simulink library "sm_wheel_loader_lib"  (R2025a)
settings: Solver=VariableStepAuto  StartTime=0.0  StopTime=10.0  RelTol=1e-3
undefined symbols (not defined in the file): AToTOrificeVector, BiPOrificeVector, boomHEArea, boomREArea, BToTOrificeVector, fluids, GRake, GToothL, GToothR, HMPST, HydFcnParams, logLoad, Position, PToAOrificeVector, PToBOrificeVector, RakeL, RakeR, testInput, Wheel_Loader, X, Y, Z
libraries: sm_lib x694, fl_lib x183, nesl_utility x74, SimscapeFluids_lib x62, sdl_lib x25, cvt_components_lib x25, simulink_extras x5, $bdroot x4, wheel_loader_contact_lib x4, ee_lib x2, SignalEditorBlockLib x1, batteryecm_lib x1
(part 2 of 26)

== system sm_wheel_loader_lib/Engine Generic ==
  EngCtrl : Inport
  Acc to I Gain : Lookup_n-D  NumberOfTableDimensions=1  BreakpointsForDimension1=[-2 -1 0 1 2]  Table=[25 25 15 15 15]  InternalRulePriority=Speed  RndMeth=Simplest
  Acc to P Gain : Lookup_n-D  NumberOfTableDimensions=1  BreakpointsForDimension1=[-2 -1 0 1 2]  Table=[50 50 15 15 15]  InternalRulePriority=Speed  RndMeth=Simplest
  Add : Sum  Inputs=+-
  Bus Creator : BusCreator  Inputs=2
  Bus Selector : BusSelector  OutputSignals=CmdEngSpd(RPM),CmdSpdRate
  Generic Engine : sdl_lib/Engines & Motors/Generic Engine  input_type=sdl.enum.GenericEngineInputType.TorqueCommand  model_parameterization=sdl.enum.engineParameterization.torque  engine_type=sdl.enum.engineType.SI  Trq_max=380 N*m  w_Trq_max=4300 rpm  P_max=230 kW  w_P_max=6858 rpm  w_max=7000 rpm  w_min=500 rpm  w_tab=[HMPST.Eng.MaxTorq.SpdVec(2:end) 3000] rpm  trq_tab=[HMPST.Eng.MaxTorq.TrqVec(2:end-2) 10 10 10] N*m  pwr_tab=[10, 30, 70, 110, 165, 190, 220, 230] kW  interp_method=simscape.enum.interpolation.linear  w_thr=100 rpm  model_inertia=sdl.enum.model_inertia.on  inertia=1 kg*m^2  initial_velocity=HMPST.Eng.wTarget rpm  model_time_constant=sdl.enum.lagOffOn.off  time_constant=0.2 s  initial_normalized_throttle=0  fc_model=sdl.enum.fuel_consumption_model.FuelOff  fc_per_rev=25 mg/rev  fc_w_tab=[1000, 2000, 3000, 4000, 5000, 6000] rpm  fc_trq_tab=[0, 80, 160, 200, 240, 320, 360, 400] N*m  fc_tab=[.5, .9, 1.4, 1.6, 1.9, 2.7, 3.4, 4.4; 1, 1.7, 2.7, 3.1, 3.6, 5, 6, 7.4; 1.4, 2.7, 4, 4.8, 5.6, 7.5, 8.5, 10.5; 2, 3.6, 5.8, 6.7, 8, 10.4, 11.7, 13.3; 2.5, 4.8, 7.9, 9.4, 10.8, 14, 16.2, 18.6; 3.1, 6, 10.3, 11.9, 13.8, 18.4, 22, 26.5] g/s  bmep_tab=[0, 250, 500, 625, 750, 1000, 1150, 1250] kPa  bsfc_tab=[410, 380, 300, 280, 270, 290, 320, 380; 410, 370, 290, 270, 260, 270, 285, 320; 415, 380, 290, 275, 265, 270, 270, 300; 420, 390, 310, 290, 285, 280, 280, 285; 430, 410, 340, 320, 310, 300, 310, 320; 450, 430, 370, 340, 330, 330, 350, 380] g/(hr*kW)  fc_interp_method=simscape.enum.interpolation.linear  displaced_volume=400 cm^3  rev_per_cycle=2  idle_speed=false  idle_speed_reference=1000 rpm  tau_controller=1 s  idle_w_thr=1 rpm  redline=false  redline_speed=5000 rpm  tau_redline=1 s  redline_w_thr=1 rpm
      settings: InternalSimscapePortConfiguration="{\"Bottom\":[],\"Left\":[{\"id\":\"TrqCmd\",\"label\":\"Trq\",\"type\":\"input\"},{\"id\":\"B\",\"label\":\"B\",\"type\":\"foundation.mechanical.rotational.rotational\"}],\"Right\":[{\"id\":\"P\",\"label\":\"P\",\"type\":\"output\"},{\"id\":\"FC\",\"label\":\"FC\",\"type\":\"output\"},{\"id\":\"F\",\"label\":\"F\",\"type\":\"foundation.mechanical.rotational.rotational\"}],\"Top\":[]}"
  Mechanical Rotational Reference : fl_lib/Mechanical/Rotational Elements/Mechanical Rotational Reference
  PID Controller : slpidlib/PID Controller  Controller=PI  Form=Parallel  TimeDomain=Continuous-time  UseExternalTs=off  SampleTime=-1  IntegratorMethod=Forward Euler  FilterMethod=Forward Euler  ControllerParametersSource=external  P=15  I=10  UseKiTs=off  D=0  UseExternalDerivativeSource=off  N=100  UseFilter=on  TunerSelectOption=Transfer Function Based (PID Tuner App)  InitialConditionSource=internal  InitialConditionForIntegrator=0  InitialConditionForFilter=0  DifferentiatorICPrevScaledInput=0  ExternalReset=none  TrackingMode=on  Kt=100  LimitOutput=off  SatLimitsSource=internal  UpperSaturationLimit=inf  LowerSaturationLimit=-inf  LinearizeAsGain=on  AntiWindupMode=none  Kb=1  LimitIntegrator=off  UpperIntegratorSaturationLimit=inf  LowerIntegratorSaturationLimit=-inf  POutMin=[]  POutMax=[]  IOutMin=[]  IOutMax=[]  DOutMin=[]  DOutMax=[]  NOutMin=[]  NOutMax=[]  SumOutMin=[]  SumOutMax=[]  SaturationOutMin=[]  SaturationOutMax=[]  PParamMin=[]  PParamMax=[]  IParamMin=[]  IParamMax=[]  DParamMin=[]  DParamMax=[]  NParamMin=[]  NParamMax=[]  KbParamMin=[]  KbParamMax=[]  KtParamMin=[]  KtParamMax=[]  KbOutMin=[]  KbOutMax=[]  KtOutMin=[]  KtOutMax=[]  IntegratorOutMin=[]  IntegratorOutMax=[]  FilterOutMin=[]  FilterOutMax=[]  SumI1OutMin=[]  SumI1OutMax=[]  SumI2OutMin=[]  SumI2OutMax=[]  SumI3OutMin=[]  SumI3OutMax=[]  SumI4OutMin=[]  SumI4OutMax=[]  SumDOutMin=[]  SumDOutMax=[]  DifferentiatorOutMin=[]  DifferentiatorOutMax=[]  FilterDiffOutCoefMin=[]  FilterDiffOutCoefMax=[]  ReciprocalOutMin=[]  ReciprocalOutMax=[]  SumDenOutMin=[]  SumDenOutMax=[]  SumNumOutMin=[]  SumNumOutMax=[]  DivideOutMin=[]  DivideOutMax=[]  UdiffTsProdOutMin=[]  UdiffTsProdOutMax=[]  NTsProdOutMin=[]  NTsProdOutMax=[]  UintegralTsProdOutMin=[]  UintegralTsProdOutMax=[]  UngainTsProdOutMin=[]  UngainTsProdOutMax=[]  ClampingZeroOutDataTypeStr=Inherit: Inherit via back propagation  ClampingZeroOutMin=[]  ClampingZeroOutMax=[]  FilterDenConstantOutDataTypeStr=Inherit: Inherit via back propagation  FilterDenConstantOutMin=[]  FilterDenConstantOutMax=[]  PCopyOutDataTypeStr=Inherit: Inherit via back propagation  PCopyOutMin=[]  PCopyOutMax=[]  NCopyOutDataTypeStr=Inherit: Inherit via back propagation  NCopyOutMin=[]  NCopyOutMax=[]  IntegratorContinuousStateAttributes=''  IntegratorStateMustResolveToSignalObject=off  IntegratorRTWStateStorageClass=Auto  FilterContinuousStateAttributes=''  FilterStateMustResolveToSignalObject=off  FilterRTWStateStorageClass=Auto  ParallelPVariant=ExternalParameters  IdealPVariant=Disabled  IVariant=ExternalParameters  DVariant=Disabled  IntegratorVariant=Continuous  SatVariant=Disabled  AWVariant=Passthrough  PCopyVariant=Disabled  TRVariant=Enabled  FdbkBlocksVariant=Forward  IdealPFdbkVariant=Disabled  SatFdbkVariant=Disabled  DerivativeFilterVariant=Disabled  NVariant=Disabled  NCopyVariant=Disabled_SignalSpec  FilterICVariant=Disabled  IntegratorICVariant=InternalICs  ExternalResetVariant=Disabled  TRSumVariant=TrackingMode  SumFdbkVariant=Disabled  SumVariant=Sum_PI  TsampFilterVariant=InternalTs  TsampNgainVariant=Passthrough  TsampIntegralVariant=Disabled_SignalSpec  ExternalSaturationOutDataTypeStr=Inherit: Same as second input  DerivativeSourceVariant=Disabled  PreIntVariant=InternalPreInt
  Simulink-PS Converter : nesl_utility/Simulink-PS Converter  PhysicalDomain=network_engine_domain  SubClassName=ps_input  LeftPortType=input  RightPortType=output  PseudoPeriodic=off  Frequencies=[]  NoiseDistribution=none  NoiseParameters=[]  Unit=1  AffineConversion=off  FilteringAndDerivatives=provide  SimscapeFilterOrder=1  InputFilterTimeConstant=0.001  UdotUserProvided=0
  Speed Sensor : Subsystem
  Subsystem : Subsystem
      settings: PortSchema="{\"entries\":[{\"content\":{\"sides\":[{\"content\":{\"connectorIds\":[\"LConn1\"]},\"type\":\"ConnectorPlacement.EquallySpacedRectSide\",\"uuid\":\"5a764f16-cafe-4867-b916-6b4e7e02daa5\"},{\"content\":{\"connectorIds\":[\"RConn1\"],\"side\":\"RIGHT\"},\"type\":\"ConnectorPlacement.EquallySpacedRectSide\",\"uuid\":\"8ceee8ac-f09f-4a1d-836f-79964ce3b2d4\"},{\"content\":{\"connectorIds\":[\"Out1\"],\"side\":\"TOP\"},\"type\":\"ConnectorPlacement.EquallySpacedRectSide\",\"uuid\":\"effcec0c-0a3a-409b-822c-5f5bf6cd9579\"}]},\"type\":\"ConnectorPlacement.EquallySpacedConnector\",\"uuid\":\"cbc631ce-3260-4296-836f-4219c3ba8d3a\"}],\"packageUris\":[\"http://schema.mathworks.com/mf0/Connector/R2020b\"],\"version\":\"1.0\"}"
  Transfer Fcn (with initial outputs) : simulink_extras/Additional Linear/Transfer Fcn (with initial outputs)  N=[1]  D="[0.1  1]"  Y0=HMPST.Eng.wTarget  U0=0
  Trq Lim Upper : Lookup_n-D  NumberOfTableDimensions=1  BreakpointsForDimension1=HMPST.Eng.MaxTorq.SpdVec  Table=HMPST.Eng.MaxTorq.TrqVec  ExtrapMethod=Clip  InternalRulePriority=Speed  RndMeth=Simplest
  Shaft : PMIOPort  Side=Right
  EngFbk : Outport
  Out Bus Element : Outport  Port=2  PortName=m  Element=w.cmd
  Out Bus Element1 : Outport  Port=2  PortName=m  Element=w.meas
  Out Bus Element2 : Outport  Port=2  PortName=m  Element=trq.limUp
  Out Bus Element3 : Outport  Port=2  PortName=m  Element=trq.meas
  Out Bus Element4 : Outport  Port=2  PortName=m  Element=trq.Cmd
  wires:
  Bus Creator/1 -> EngFbk/1
  Bus Selector/1 -> Transfer Fcn (with initial outputs)/1  "<CmdEngSpd(RPM)>"
  EngCtrl/1 -> Bus Selector/1
  Bus Selector/2 -> Acc to P Gain/1, Acc to I Gain/1  "<CmdSpdRate>"
  Acc to P Gain/1 -> PID Controller/2
  Acc to I Gain/1 -> PID Controller/3
  Speed Sensor/1(w (rpm)) -> Add/2, Out Bus Element1/1, Trq Lim Upper/1, Bus Creator/2  "ActuEngSpd(RPM)"
  Trq Lim Upper/1 -> Out Bus Element2/1  "UL_Trq"
  PID Controller/1 -> Out Bus Element4/1, PID Controller/4, Bus Creator/1, Simulink-PS Converter/1  "ActuEngTrq(Nm)"
  Transfer Fcn (with initial outputs)/1 -> Add/1, Out Bus Element/1  "Cmd Speed (RPM)"
  Add/1 -> PID Controller/1
  Subsystem/1(m) -> Out Bus Element3/1
  connections:
  Speed Sensor/LConn1 -- Subsystem/LConn1 -- Generic Engine/RConn3
  Mechanical Rotational Reference/LConn1 -- Generic Engine/LConn2
  Simulink-PS Converter/RConn1 -- Generic Engine/LConn1
  Shaft/RConn1 -- Subsystem/RConn1

== system sm_wheel_loader_lib/Hydrostatic ==
  note: Convert transmission ratio to swash plate ratio
  BusElementIn : Inport  PortName=Ctrl  Element=MBCtrl
  BusElementIn1 : Inport  PortName=Ctrl  Element=ratio
  BusElementIn2 : Inport  PortName=Ctrl  Element=CmdVehSpdDir
  Bearing Friction : sdl_lib/Couplings & Drives/Springs & Dampers/Rotational Damper  D=HMPST.Bearing.dVisc N*m*s/rad  thermal_port=simscape.enum.thermaleffects.omit  thermal_mass=50 kJ/K  temperature_specify=off  temperature_priority=High  temperature=300 K  temperature_nominal_specify=off  temperature_nominal_value=1  temperature_nominal_unit=K
  Brake Out : cvt_components_lib/Brake  bore=HMPST.Brake.cylBore  brkwy_vel=HMPST.Brake.vBrk  mu_static=HMPST.Brake.muSta  mu_coulomb=HMPST.Brake.muKin  n_pads=HMPST.Brake.numPads  r_mean=HMPST.Brake.rPad  visc_coef=HMPST.Brake.dVisc  logic2pressure=HMPST.Brake.logic2Press  ts_filt=HMPST.Brake.tsFilt
  Constant : Constant  Value=0
  Constant1 : Constant  Value=HMPST.Eng.wTarget/HMPST.HydroUnit.Pump.SpeedLimit
  Constant2 : Constant  Value=HMPST.HydroUnit.Motor.Disp/HMPST.HydroUnit.Pump.Disp
  Gain : Gain  Gain=-1
  Gears HS In : $bdroot/CVT Power Split Hydromechanical/Gears HS In  SystemSampleTime=-1  VariantActivationTime=update diagram  EmptyChoice=off  PassThrough=off  PassThroughVariantControl=(default)  EmptyChoiceVariantControl=(default)  AllowFlexibleInterface=on  Latency=0  AutoFrameSizeCalculation=off
  Hydrostatic : $bdroot/CVT Power Split Hydromechanical/Hydrostatic  pumpNomDisp=HMPST.HydroUnit.Pump.Disp  motorNomDisp=HMPST.HydroUnit.Motor.Disp  pumpNomSpd=HMPST.HydroUnit.Pump.SpeedLimit  motorNomSpd=HMPST.HydroUnit.Motor.wNominal  pumpNomVolEff=HMPST.HydroUnit.Pump.volEffNominal  motorNomVolEff=HMPST.HydroUnit.Motor.volEffNominal  pumpNomMechEff=HMPST.HydroUnit.Pump.mechEffNominal  motorNomMechEff=HMPST.HydroUnit.Motor.mechEffNominal  pumpNomPressGain=HMPST.HydroUnit.Pump.prGainNominal  motorNomPressDrop=HMPST.HydroUnit.Motor.prDropNominal  p_crack_differential=HMPST.HydroUnit.ChkV.pDiffCrack  press_max_differential=HMPST.HydroUnit.ChkV.pDiffMax  chkv_area_max=HMPST.HydroUnit.ChkV.aMax  chkv_area_leak=HMPST.HydroUnit.ChkV.aLeak  p_set_differential=HMPST.HydroUnit.PrV.pDiffSet  p_range=HMPST.HydroUnit.PrV.pRange  prv_area_max=HMPST.HydroUnit.PrV.aMax  prv_area_leak=HMPST.HydroUnit.PrV.aLeak  pipeLen=HMPST.HydroUnit.Pipes.len  pipeAreaGeo=HMPST.HydroUnit.Pipes.aGeom  pipeAreaHydr=HMPST.HydroUnit.Pipes.aHydr  chgPumpNomDisp=HMPST.HydroUnit.ChargePump.Disp  chgPumpNomMechEff=HMPST.HydroUnit.ChargePump.mechEffNominal  chgPumpNomPressGain=HMPST.HydroUnit.ChargePump.prGainNominal  chgPumpNomSpd=HMPST.HydroUnit.ChargePump.wNominal  chgPumpNomVolEff=HMPST.HydroUnit.ChargePump.volEffNominal  chgPumpChkvAleak=HMPST.HydroUnit.ChargePumpPrV.aLeak  chgPumpChkvAmax=HMPST.HydroUnit.ChargePumpPrV.aMax  chgPumpChkvPdiff=HMPST.HydroUnit.ChargePumpPrV.pDiffSet  chgPumpChkvPrange=HMPST.HydroUnit.ChargePumpPrV.pRange
  Mechanical Rotational Reference : fl_lib/Mechanical/Rotational Elements/Mechanical Rotational Reference
  Product : Product
  Product1 : Product  Inputs=3
  Sensor wIn : $bdroot/CVT Abstract/Sensor wIn  SystemSampleTime=-1  VariantActivationTime=update diagram  EmptyChoice=off  PassThrough=off  PassThroughVariantControl=(default)  EmptyChoiceVariantControl=(default)  AllowFlexibleInterface=on  Latency=0  AutoFrameSizeCalculation=off
  Sensor wOut : $bdroot/CVT Abstract/Sensor wOut  SystemSampleTime=-1  VariantActivationTime=update diagram  EmptyChoice=off  PassThrough=off  PassThroughVariantControl=(default)  EmptyChoiceVariantControl=(default)  AllowFlexibleInterface=on  Latency=0  AutoFrameSizeCalculation=off
  E : PMIOPort  Side=Left
  D : PMIOPort  Port=2  Side=Right
  Out Bus Element : Outport  PortName=m  Element=wIn
  Out Bus Element11 : Outport  PortName=m  Element=OutputShaft
  Out Bus Element12 : Outport  PortName=m  Element=P_acc
  wires:
  BusElementIn/1 -> Brake Out/1
  BusElementIn1/1 -> Product/1
  BusElementIn2/1 -> Product/2
  Product/1 -> Gain/1
  Sensor wOut/1 -> Out Bus Element11/1
  Sensor wIn/1 -> Out Bus Element/1
  Gain/1 -> Product1/1
  Product1/1 -> Hydrostatic/1
  Constant1/1 -> Product1/2
  Constant2/1 -> Product1/3
  Constant/1 -> Out Bus Element12/1  "P_acc"
  connections:
  E/RConn1 -- Gears HS In/LConn1
  D/RConn1 -- Sensor wOut/LConn1 -- Brake Out/RConn1 -- Bearing Friction/LConn1 -- Hydrostatic/RConn1
  Hydrostatic/LConn1 -- Gears HS In/RConn3
  Sensor wIn/LConn1 -- Gears HS In/RConn1
  Bearing Friction/RConn1 -- Mechanical Rotational Reference/LConn1

== system sm_wheel_loader_lib/Tires and Body 1D ==
  PS-Simulink Converter : nesl_utility/PS-Simulink Converter  PhysicalDomain=network_engine_domain  SubClassName=ps_output  LeftPortType=input  RightPortType=output  PseudoPeriodic=off  Frequencies=[]  VectorFormat=inherit  Unit=km/hr  AffineConversion=off
  Tire FL : sdl_lib/Tires & Vehicles/Tire (Magic Formula)  parameterization=sdl.enum.magic_tire_model.peak  F_z1=HMPST.TireMF1D.FA.fZrated N  F_x1=HMPST.TireMF1D.FA.fXrated N  kappa1=HMPST.TireMF1D.FA.slipRated  B_m=10  C_m=1.9  D_m=1  E_m=0.97  fz0=4000 N  p_Cx=1.685  p_Dx=[1.21, -.037]  p_Ex=[.344, .095, -.02, 0]  p_Kx=[21.51, -.163, .245]  p_Hx=[-.002, .002]  p_Vx=[0, 0]  rolling_radius_model=sdl.enum.RollingRadiusParameterization.Constant  r_e=HMPST.Tire.Rad m  r_0=0.3 m  breff=8.39  dreff=0.26  freff=0.074  q_re0=0.99  q_v1=0.008  longvl=17 m/s  cz=5e5 N/m  model_resistance=true  resistance_model=sdl.enum.rollingResistanceParameterization.constant  coeff=HMPST.TireMF1D.FA.rollingR.coeff  p_tire=250e3 Pa  alpha=-0.003  beta=0.97  coeff_a=84e-4  coeff_b=6.2e-4 s/m  coeff_c=1.6e-4 s^2/m^2  p_tire0=240e3 Pa  fz0_resistance=4000 N  vH0=16 m/s  q_Sy=[.0082, 0, .0014, .001, 0, 0, 1.08, -.5]  v_thr=HMPST.TireMF1D.FA.rollingR.vth m/s  enable_scaling_coefficients=false  lfzO=1  lcx=1  lmux=1  lex=1  lkx=1  lhx=1  lvx=1  lmy=1  model_compliance=sdl.enum.compliance.off  stiffness=1e6 N/m  damping=1000 N*s/m  model_inertia=sdl.enum.model_inertia.off  inertia=1 kg*m^2  initial_velocity=0 rad/s  vxlow=1 m/s  v_tr_thr=0.1 m/s  kpumin=-1.5  kpumax=1.5
  Tire FR : sdl_lib/Tires & Vehicles/Tire (Magic Formula)  parameterization=sdl.enum.magic_tire_model.peak  F_z1=HMPST.TireMF1D.FA.fZrated N  F_x1=HMPST.TireMF1D.FA.fXrated N  kappa1=HMPST.TireMF1D.FA.slipRated  B_m=10  C_m=1.9  D_m=1  E_m=0.97  fz0=4000 N  p_Cx=1.685  p_Dx=[1.21, -.037]  p_Ex=[.344, .095, -.02, 0]  p_Kx=[21.51, -.163, .245]  p_Hx=[-.002, .002]  p_Vx=[0, 0]  rolling_radius_model=sdl.enum.RollingRadiusParameterization.Constant  r_e=HMPST.Tire.Rad m  r_0=0.3 m  breff=8.39  dreff=0.26  freff=0.074  q_re0=0.99  q_v1=0.008  longvl=17 m/s  cz=5e5 N/m  model_resistance=true  resistance_model=sdl.enum.rollingResistanceParameterization.constant  coeff=HMPST.TireMF1D.FA.rollingR.coeff  p_tire=250e3 Pa  alpha=-0.003  beta=0.97  coeff_a=84e-4  coeff_b=6.2e-4 s/m  coeff_c=1.6e-4 s^2/m^2  p_tire0=240e3 Pa  fz0_resistance=4000 N  vH0=16 m/s  q_Sy=[.0082, 0, .0014, .001, 0, 0, 1.08, -.5]  v_thr=HMPST.TireMF1D.FA.rollingR.vth m/s  enable_scaling_coefficients=false  lfzO=1  lcx=1  lmux=1  lex=1  lkx=1  lhx=1  lvx=1  lmy=1  model_compliance=sdl.enum.compliance.off  stiffness=1e6 N/m  damping=1000 N*s/m  model_inertia=sdl.enum.model_inertia.off  inertia=1 kg*m^2  initial_velocity=0 rad/s  vxlow=1 m/s  v_tr_thr=0.1 m/s  kpumin=-1.5  kpumax=1.5
  Tire RL : sdl_lib/Tires & Vehicles/Tire (Magic Formula)  parameterization=sdl.enum.magic_tire_model.peak  F_z1=HMPST.TireMF1D.RA.fZrated N  F_x1=HMPST.TireMF1D.RA.fXrated N  kappa1=HMPST.TireMF1D.RA.slipRated  B_m=10  C_m=1.9  D_m=1  E_m=0.97  fz0=4000 N  p_Cx=1.685  p_Dx=[1.21, -.037]  p_Ex=[.344, .095, -.02, 0]  p_Kx=[21.51, -.163, .245]  p_Hx=[-.002, .002]  p_Vx=[0, 0]  rolling_radius_model=sdl.enum.RollingRadiusParameterization.Constant  r_e=HMPST.Tire.Rad m  r_0=0.3 m  breff=8.39  dreff=0.26  freff=0.074  q_re0=0.99  q_v1=0.008  longvl=17 m/s  cz=5e5 N/m  model_resistance=true  resistance_model=sdl.enum.rollingResistanceParameterization.constant  coeff=HMPST.TireMF1D.RA.rollingR.coeff  p_tire=250e3 Pa  alpha=-0.003  beta=0.97  coeff_a=84e-4  coeff_b=6.2e-4 s/m  coeff_c=1.6e-4 s^2/m^2  p_tire0=240e3 Pa  fz0_resistance=4000 N  vH0=16 m/s  q_Sy=[.0082, 0, .0014, .001, 0, 0, 1.08, -.5]  v_thr=HMPST.TireMF1D.RA.rollingR.vth m/s  enable_scaling_coefficients=false  lfzO=1  lcx=1  lmux=1  lex=1  lkx=1  lhx=1  lvx=1  lmy=1  model_compliance=sdl.enum.compliance.off  stiffness=1e6 N/m  damping=1000 N*s/m  model_inertia=sdl.enum.model_inertia.off  inertia=1 kg*m^2  initial_velocity=0 rad/s  vxlow=1 m/s  v_tr_thr=0.1 m/s  kpumin=-1.5  kpumax=1.5
  Tire RR : sdl_lib/Tires & Vehicles/Tire (Magic Formula)  parameterization=sdl.enum.magic_tire_model.peak  F_z1=HMPST.TireMF1D.RA.fZrated N  F_x1=HMPST.TireMF1D.RA.fXrated N  kappa1=HMPST.TireMF1D.RA.slipRated  B_m=10  C_m=1.9  D_m=1  E_m=0.97  fz0=4000 N  p_Cx=1.685  p_Dx=[1.21, -.037]  p_Ex=[.344, .095, -.02, 0]  p_Kx=[21.51, -.163, .245]  p_Hx=[-.002, .002]  p_Vx=[0, 0]  rolling_radius_model=sdl.enum.RollingRadiusParameterization.Constant  r_e=HMPST.Tire.Rad m  r_0=0.3 m  breff=8.39  dreff=0.26  freff=0.074  q_re0=0.99  q_v1=0.008  longvl=17 m/s  cz=5e5 N/m  model_resistance=true  resistance_model=sdl.enum.rollingResistanceParameterization.constant  coeff=HMPST.TireMF1D.RA.rollingR.coeff  p_tire=250e3 Pa  alpha=-0.003  beta=0.97  coeff_a=84e-4  coeff_b=6.2e-4 s/m  coeff_c=1.6e-4 s^2/m^2  p_tire0=240e3 Pa  fz0_resistance=4000 N  vH0=16 m/s  q_Sy=[.0082, 0, .0014, .001, 0, 0, 1.08, -.5]  v_thr=HMPST.TireMF1D.RA.rollingR.vth m/s  enable_scaling_coefficients=false  lfzO=1  lcx=1  lmux=1  lex=1  lkx=1  lhx=1  lvx=1  lmy=1  model_compliance=sdl.enum.compliance.off  stiffness=1e6 N/m  damping=1000 N*s/m  model_inertia=sdl.enum.model_inertia.off  inertia=1 kg*m^2  initial_velocity=0 rad/s  vxlow=1 m/s  v_tr_thr=0.1 m/s  kpumin=-1.5  kpumax=1.5
  Vehicle Body : sdl_lib/Tires & Vehicles/Vehicle Body  mass=HMPST.Veh.Mass kg  n_w=2  x_f=HMPST.Veh.CG.FA2CGx m  x_r=HMPST.Veh.CG.RA2CGx m  y_c=HMPST.Veh.CG.FA2CGz m  mass_var=simscape.enum.onoff.off  g=9.81 m/s^2  liftoff_warning=simscape.enum.onoff.off  area=3 m^2  Cd_var=false  Cd=0.4  rho=1.18 kg/m^3  model_pitch=simscape.enum.onoff.off  inertia=4000 kg*m^2  suspension_model=sdl.enum.linearTLU.linear  k_f=1e4 N/m  b_f=1e4 N*s/m  k_r=1e4 N/m  b_r=1e4 N*s/m  k_f_TLU=[-2000, -1000, 0, 1000, 2000] N  x_f_TLU=[-.4, -.2, 0, .2, .4] m  b_f_TLU=[-200, -100, 0, 100, 200] N  v_f_TLU=[-4, -2, 0, 2, 4] m/s  k_r_TLU=[-2000, -1000, 0, 1000, 2000] N  x_r_TLU=[-.4, -.2, 0, .2, .4] m  b_r_TLU=[-200, -100, 0, 100, 200] N  v_r_TLU=[-4, -2, 0, 2, 4] m/s  interp_method=simscape.enum.interpolation.linear  extrap_method=simscape.enum.extrapolation.linear  model_hardstop=simscape.enum.onoff.off  upper_bound_f=.25 m  lower_bound_f=-.25 m  stop_k_f=1e6 N/m  stop_b_f=150 N*s/m  upper_bound_r=.25 m  lower_bound_r=-.25 m  stop_k_r=1e6 N/m  stop_b_r=150 N*s/m  initial_pitch=0 rad  initial_pitch_rate=0 rad/s  v_specify=off  v_priority=High  v=0 m/s  v_nominal_specify=off  v_nominal_value=1  v_nominal_unit=m/s
      settings: InternalSimscapePortConfiguration="{\"Bottom\":[{\"id\":\"NR\",\"label\":\"NR\",\"type\":\"output\"},{\"id\":\"NF\",\"label\":\"NF\",\"type\":\"output\"},{\"id\":\"beta\",\"label\":\"beta\",\"type\":\"input\"}],\"Left\":[{\"id\":\"H\",\"label\":\"H\",\"type\":\"foundation.mechanical.translational.translational\"}],\"Right\":[],\"Top\":[{\"id\":\"V\",\"label\":\"V\",\"type\":\"output\"},{\"id\":\"wind\",\"label\":\"W\",\"type\":\"input\"}]}"
  FL : PMIOPort  Side=Left
  RL : PMIOPort  Port=2  Side=Left
  FR : PMIOPort  Port=3  Side=Right
  RR : PMIOPort  Port=4  Side=Right
  v : Outport
  wires:
  PS-Simulink Converter/1 -> v/1
  connections:
  Vehicle Body/RConn1 -- Tire RR/LConn1 -- Tire RL/LConn1
  Vehicle Body/LConn2 -- PS-Simulink Converter/LConn1
  Tire FL/RConn2 -- Tire FR/RConn2 -- Tire RR/RConn2 -- Tire RL/RConn2 -- Vehicle Body/LConn1
  Tire RR/LConn2 -- RR/RConn1
  Vehicle Body/RConn2 -- Tire FR/LConn1 -- Tire FL/LConn1
  Tire FL/LConn2 -- FL/RConn1
  Tire FR/LConn2 -- FR/RConn1
  Tire RL/LConn2 -- RL/RConn1

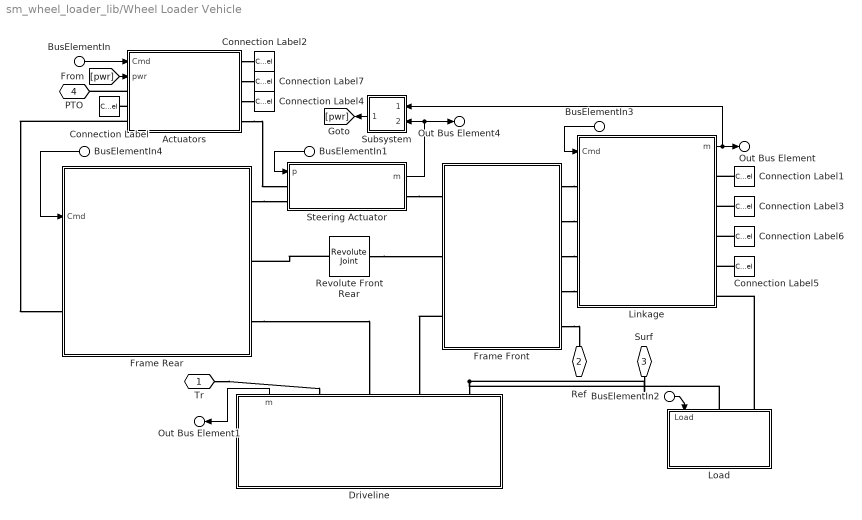
== system sm_wheel_loader_lib/Wheel Loader Vehicle ==
  BusElementIn{,1,3..4} (4 alike) : Inport  PortName=Cmd
  BusElementIn2 : Inport  PortName=Cmd  Element=Actuator.InertiaLoad
  Actuators : Subsystem  Variant=on  VariantControlMode=label  VariantControl=Actuators  LabelModeActiveChoice=Ideal  mask{popup_impl=Bucket}
      mask prompts: popup_impl "Implement"
      mask init:
      | if(strcmp(get_param(gcb,'popup_impl'),'Bucket'))
      |     set_param([gcb '/Hydraulic'],'popup_impl','Bucket');
      | else
      |     set_param([gcb '/Hydraulic'],'popup_impl','Grapple');
      | end
      settings: AttributesFormatString=%<LabelModeActiveChoice>, %<popup_impl>
      mask TypeOptions popup_impl: Bucket | Grapple
  Connection Label : ConnectionLabel  Label=Tilt
  Connection Label1 : ConnectionLabel  Label=Tilt
  Connection Label2 : ConnectionLabel  Label=LiftL
  Connection Label3 : ConnectionLabel  Label=LiftL
  Connection Label4 : ConnectionLabel  Label=Impl
  Connection Label5 : ConnectionLabel  Label=Impl
  Connection Label6 : ConnectionLabel  Label=LiftR
  Connection Label7 : ConnectionLabel  Label=LiftR
  Driveline : Subsystem  mask{popup_driveline_model=Driveline 1D, popup_driveJointF=CV Joint, popup_driveJointR=CV Joint, popup_contact=Sphere}
      mask prompts: popup_driveline_model "Driveline Model"; popup_driveJointF "Driveline Joint (front)"; popup_driveJointR "Driveline Joint (rear)"; popup_contact "Contact Geometry"
      mask init:
      | if(strcmp(get_param(gcb,'popup_driveline_model'),'Driveline 1D'))
      |     set_param([gcb '/Driveline'],'LabelModeActiveChoice','Driveline_1D')
      | else
      |     set_param([gcb '/Driveline'],'LabelModeActiveChoice','Driveline_3D')
      |     set_param([gcb '/Driveline'],'popup_driveJointF',...
      |         get_param(gcb,'popup_driveJointF'));
      |     set_param([gcb '/Driveline'],'popup_driveJointR',...
      |         get_param(gcb,'popup_driveJointR'));
      | end
      settings: AttributesFormatString=%<popup_driveline_model>
      mask TypeOptions popup_driveline_model: Driveline 1D | Driveline 3D
      mask TypeOptions popup_driveJointF: CV Joint | U Joint
      mask TypeOptions popup_driveJointR: CV Joint | U Joint
      mask TypeOptions popup_contact:
      | Ground
      | Contact FL/popup_contact | Ground
      | Contact FR/popup_contact | Ground
      | Contact RL/popup_contact | Ground
      | Contact RR/popup_contact
      mask Display: image('sm_wheel_loader_vehicle_wheelsDriveline3D_IMAGE.png');
  Frame Front : Subsystem
      mask Display: image('sm_wheel_loader_vehicle_frameFront_IMAGE.png')
  Frame Rear : Subsystem
      mask Display: image('sm_wheel_loader_vehicle_frameRear_IMAGE.png')
  Linkage : Subsystem  mask{popup_impl=Bucket, popup_actuator_model=Position}
      mask prompts: popup_impl "Implement"; popup_actuator_model "Actuator Mode"
      mask init:
      | set_param([gcb '/Implement'],'LabelModeActiveChoice',get_param(gcb, ...
      |     'popup_impl'));
      settings: AttributesFormatString=%<popup_impl>, %<popup_actuator_model>
      mask TypeOptions popup_impl: Bucket | Grapple
      mask TypeOptions popup_actuator_model: Implement/popup_actuator_model | Lift Actuator L/popup_actuator_model | Lift Actuator R/popup_actuator_model | ZBar/popup_actuator_model
      mask Display:
      | if(strcmp(get_param(gcb,'popup_impl'),'Grapple'))
      |     image('sm_wheel_loader_vehicle_linkageGrapple_IMAGE.png')
      | else
      |     image('sm_wheel_loader_vehicle_linkageBucket_IMAGE.png')
      | end
  Load : Subsystem  Variant=on  VariantControlMode=label  VariantControl=Choice  LabelModeActiveChoice=None  mask{base_pos=logLoad.YCycle.basePos, base_ori=logLoad.YCycle.baseOri, bin_pos=logLoad.YCycle.binPos, bin_ori=logLoad.YCycle.binOri}
      mask prompts: base_pos "Log Base Position [x y z] (m)"; base_ori "Log Base Orientation (deg)"; bin_pos "Bin Position [x y z] (m)"; bin_ori "Bin Orientation (deg)"
      settings: AttributesFormatString=%<LabelModeActiveChoice>
  Revolute Front Rear : sm_lib/Joints/Revolute Joint  JointMode=Normal  CompositeWrenchDir=FollowerOnBase  CompositeWrenchFrame=BaseFrame  SenseConstraintForce=off  SenseConstraintTorque=off  SenseTotalForce=off  SenseTotalTorque=off  PositionTargetSpecify=off  PositionTargetPriority=High  PositionTargetValue=0  PositionTargetValueUnits=deg  VelocityTargetSpecify=off  VelocityTargetPriority=High  VelocityTargetValue=0  VelocityTargetValueUnits=deg/s  EquilibriumPosition=0  EquilibriumPositionUnits=deg  SpringStiffness=0  SpringStiffnessUnits=N*m/deg  DampingCoefficient=0  DampingCoefficientUnits=N*m/(rad/s)  LowerLimitSpecify=off  LowerLimitBound=-90  LowerLimitBoundUnits=deg  LowerLimitStiffness=1e4  LowerLimitStiffnessUnits=N*m/deg  LowerLimitDamping=10  LowerLimitDampingUnits=N*m/(deg/s)  LowerLimitTransitionRegionWidth=0.1  LowerLimitTransitionRegionWidthUnits=deg  UpperLimitSpecify=off  UpperLimitBound=90  UpperLimitBoundUnits=deg  UpperLimitStiffness=1e4  UpperLimitStiffnessUnits=N*m/deg  UpperLimitDamping=10  UpperLimitDampingUnits=N*m/(deg/s)  UpperLimitTransitionRegionWidth=0.1  UpperLimitTransitionRegionWidthUnits=deg  TorqueActuationMode=NoTorque  MotionActuationMode=ComputedMotion  SensePosition=off  SenseVelocity=off  SenseAcceleration=off  SenseTorqueForce=off  SenseLowerLimitTorqueForce=off  SenseUpperLimitTorqueForce=off
  Steering Actuator : Subsystem  mask{popup_actuator_model=Position}
      mask prompts: popup_actuator_model "Actuation Mode"
      mask init:
      | if(strcmp(get_param(gcb,'popup_actuator_model'),'Shaft'))
      |     set_param([gcb '/Actuator'],'LabelModeActiveChoice','Shaft')
      | else
      |     set_param([gcb '/Actuator'],'LabelModeActiveChoice','Position')
      | end
      mask TypeOptions popup_actuator_model: Shaft | Position
      mask Display:
      | if(strcmp(get_param(gcb,'popup_actuator_model'),'Position'))
      |     image('sm_wheel_loader_actuator_intfPosition_IMAGE.png')
      | else
      |     image('sm_wheel_loader_actuator_intfShaft_IMAGE.png')
      | end
  Subsystem : Subsystem
  Tr : PMIOPort  Side=Left
  Ref : PMIOPort  Port=2  Side=Right
  Surf : PMIOPort  Port=3  Side=Right
  PTO : PMIOPort  Port=4  Side=Left
  Out Bus Element : Outport  PortName=m  Element=Linkage
  Out Bus Element4 : Outport  PortName=m  Element=Steer
  Out Bus Element1 : Outport  PortName=m  Element=Driveline
  wires:
  Driveline/1(m) -> Out Bus Element1/1
  BusElementIn2/1 -> Load/1(Load)
  Steering Actuator/1(m) -> Subsystem/2(Str), Out Bus Element4/1
  Linkage/1(m) -> Subsystem/1(Link), Out Bus Element/1
  BusElementIn/1 -> Actuators/1(Cmd)
  BusElementIn1/1 -> Steering Actuator/1(p)
  BusElementIn3/1 -> Linkage/1(Cmd)
  BusElementIn4/1 -> Frame Rear/1(Cmd)
  Subsystem/1(pwr) -> [pwr]
  [pwr] -> Actuators/2(pwr)
  connections:
  Tr/RConn1 -- Driveline/RConn1
  Frame Front/LConn3 -- Driveline/RConn3
  Frame Rear/RConn3 -- Driveline/RConn2
  Driveline/RConn4 -- Load/LConn1 -- Surf/RConn1
  Load/LConn2 -- Linkage/RConn5
  Revolute Front Rear/LConn1 -- Frame Rear/RConn2
  Revolute Front Rear/RConn1 -- Frame Front/LConn2
  Frame Front/RConn1 -- Linkage/LConn1
  Frame Front/RConn2 -- Linkage/LConn2
  Frame Front/RConn3 -- Linkage/LConn3
  Frame Front/RConn4 -- Linkage/LConn4
  Steering Actuator/RConn1 -- Frame Front/LConn1
  Frame Rear/RConn1 -- Steering Actuator/LConn2
  Frame Front/RConn5 -- Ref/RConn1
  Connection Label1/LConn1 -- Linkage/RConn1
  Connection Label3/LConn1 -- Linkage/RConn2
  Connection Label5/LConn1 -- Linkage/RConn4
  Connection Label6/LConn1 -- Linkage/RConn3
  Actuators/LConn1 -- PTO/RConn1
  Actuators/RConn1 -- Connection Label2/LConn1
  Actuators/RConn2 -- Connection Label7/LConn1
  Actuators/LConn2 -- Connection Label/LConn1
  Actuators/RConn3 -- Connection Label4/LConn1
  Actuators/RConn4 -- Steering Actuator/LConn1
  Actuators/LConn3 -- Frame Rear/LConn1

== system sm_wheel_loader_lib/CVT Abstract/Sensor wIn ==
  MRRef : fl_lib/Mechanical/Rotational Elements/Mechanical Rotational Reference
  Motion Sensor : fl_lib/Mechanical/Mechanical Sensors/Ideal Rotational Motion Sensor  reference=foundation.enum.MeasurementReference.difference  acceleration_port=false  velocity_port=true  position_port=false  wrap_angle=false  offset=0 rad
      settings: InternalSimscapePortConfiguration="{\"Bottom\":[],\"Left\":[{\"id\":\"R\",\"label\":\"R\",\"type\":\"foundation.mechanical.rotational.rotational\"}],\"Right\":[{\"id\":\"C\",\"label\":\"C\",\"type\":\"foundation.mechanical.rotational.rotational\"},{\"id\":\"W\",\"label\":\"W\",\"type\":\"output\"}],\"Top\":[]}"
  PS-Simulink Converter : nesl_utility/PS-Simulink Converter  PhysicalDomain=network_engine_domain  SubClassName=ps_output  LeftPortType=input  RightPortType=output  PseudoPeriodic=off  Frequencies=[]  VectorFormat=inherit  Unit=rpm  AffineConversion=off
  R : PMIOPort  Side=Left
  w : Outport
  wires:
  PS-Simulink Converter/1 -> w/1
  connections:
  R/RConn1 -- Motion Sensor/LConn1
  MRRef/LConn1 -- Motion Sensor/RConn1
  PS-Simulink Converter/LConn1 -- Motion Sensor/RConn2

== system sm_wheel_loader_lib/CVT Abstract/Sensor wOut ==
  MRRef : fl_lib/Mechanical/Rotational Elements/Mechanical Rotational Reference
  Motion Sensor : fl_lib/Mechanical/Mechanical Sensors/Ideal Rotational Motion Sensor  reference=foundation.enum.MeasurementReference.difference  acceleration_port=false  velocity_port=true  position_port=false  wrap_angle=false  offset=0 rad
      settings: InternalSimscapePortConfiguration="{\"Bottom\":[],\"Left\":[{\"id\":\"R\",\"label\":\"R\",\"type\":\"foundation.mechanical.rotational.rotational\"}],\"Right\":[{\"id\":\"C\",\"label\":\"C\",\"type\":\"foundation.mechanical.rotational.rotational\"},{\"id\":\"W\",\"label\":\"W\",\"type\":\"output\"}],\"Top\":[]}"
  PS-Simulink Converter : nesl_utility/PS-Simulink Converter  PhysicalDomain=network_engine_domain  SubClassName=ps_output  LeftPortType=input  RightPortType=output  PseudoPeriodic=off  Frequencies=[]  VectorFormat=inherit  Unit=rpm  AffineConversion=off
  R : PMIOPort  Side=Left
  w : Outport
  wires:
  PS-Simulink Converter/1 -> w/1
  connections:
  PS-Simulink Converter/LConn1 -- Motion Sensor/RConn2
  MRRef/LConn1 -- Motion Sensor/RConn1
  R/RConn1 -- Motion Sensor/LConn1

== system sm_wheel_loader_lib/CVT Electrical/Control ==
  ratioCmd : Inport
  wOut : Inport  Port=2
  wIn : Inport  Port=3
  Control : Subsystem
  Gain : Gain  Gain=-1
  Product : Product
  Product1 : Product
  trqMot : Outport
  trqGen : Outport  Port=2
  wires:
  wOut/1 -> Control/2(wMeas)
  Product/1 -> Control/1(wCmd)
  ratioCmd/1 -> Product1/1, Product/1
  wIn/1 -> Gain/1
  Control/1(Trq) -> trqMot/1, Product1/2
  Product1/1 -> trqGen/1
  Gain/1 -> Product/2

== system sm_wheel_loader_lib/CVT Power Split Hydromechanical/Gear Kr ==
  Gear Kr : sdl_lib/Gears/Simple Gear  ratio=1  rotation_direction=3-2*(2)  friction_model=sdl.enum.gear_efficiencies_load.off  T_noload=0.1 N*m  T_nom=5 N*m  efficiency_nom=0.8  efficiency=0.995  temperature_TLU=[ 280 300 320 ] K  load_TLU=[ 1 5 10 ] N*m  efficiency_TLU=[ 0.95 0.9 0.85 ]  efficiency_TLU2=[ 0.85 0.8 0.75; 0.95 0.9 0.85; 0.85 0.8 0.7 ]  w_thr=0.01 rad/s  pwr_thr=0.001 W  enable_backlash=false  hardstop_model=simscape.enum.hardstop.smooth  backlash_distance=1e-3 mm  r_base=0.1 m  transition=1e-4 mm  backlash_stiffness=1e6 N/m  backlash_damping=1e3 N*s/m  coeff_rest=0.7  v_tol=0.001 m/s  f_tol=0 N  mu_visc=[0 0] N*m/(rad/s)  thermal_mass=50 J/K  temperature_specify=off  temperature_priority=High  temperature=300 K  temperature_nominal_specify=off  temperature_nominal_value=1  temperature_nominal_unit=K  x_backlash_specify=off  x_backlash_priority=None  x_backlash=0 mm  x_backlash_nominal_specify=off  x_backlash_nominal_value=1  x_backlash_nominal_unit=mm  f_hardstop_specify=off  f_hardstop_priority=None  f_hardstop=0 N  f_hardstop_nominal_specify=off  f_hardstop_nominal_value=1  f_hardstop_nominal_unit=N  v_backlash_specify=off  v_backlash_priority=None  v_backlash=0 m/s  v_backlash_nominal_specify=off  v_backlash_nominal_value=1  v_backlash_nominal_unit=m/s
  Inertia Kr : fl_lib/Mechanical/Rotational Elements/Inertia  inertia=1 kg*m^2  num_ports=foundation.enum.numPorts2.two  w_specify=off  w_priority=High  w=0 rad/s  w_nominal_specify=off  w_nominal_value=1  w_nominal_unit=rad/s  t_specify=off  t_priority=None  t=0 N*m  t_nominal_specify=off  t_nominal_value=1  t_nominal_unit=N*m
      settings: InternalSimscapePortConfiguration="{\"Bottom\":[],\"Left\":[{\"id\":\"I\",\"label\":\"\",\"type\":\"foundation.mechanical.rotational.rotational\"}],\"Right\":[{\"id\":\"J\",\"label\":\"\",\"type\":\"foundation.mechanical.rotational.rotational\"}],\"Top\":[]}"
  "     B" : PMIOPort  Side=Left
  "    F" : PMIOPort  Port=2  Side=Left
  connections:
  Gear Kr/RConn1 -- "    F"/RConn1
  Inertia Kr/LConn1 -- "     B"/RConn1
  Inertia Kr/RConn1 -- Gear Kr/LConn1

== system sm_wheel_loader_lib/CVT Power Split Hydromechanical/Gear Kv ==
  Gear Kv : sdl_lib/Gears/Simple Gear  ratio=1  rotation_direction=3-2*(1)  friction_model=sdl.enum.gear_efficiencies_load.off  T_noload=0.1 N*m  T_nom=5 N*m  efficiency_nom=0.8  efficiency=0.995  temperature_TLU=[ 280 300 320 ] K  load_TLU=[ 1 5 10 ] N*m  efficiency_TLU=[ 0.95 0.9 0.85 ]  efficiency_TLU2=[ 0.85 0.8 0.75; 0.95 0.9 0.85; 0.85 0.8 0.7 ]  w_thr=0.01 rad/s  pwr_thr=0.001 W  enable_backlash=false  hardstop_model=simscape.enum.hardstop.smooth  backlash_distance=1e-3 mm  r_base=0.1 m  transition=1e-4 mm  backlash_stiffness=1e6 N/m  backlash_damping=1e3 N*s/m  coeff_rest=0.7  v_tol=0.001 m/s  f_tol=0 N  mu_visc=[0 0] N*m/(rad/s)  thermal_mass=50 J/K  temperature_specify=off  temperature_priority=High  temperature=300 K  temperature_nominal_specify=off  temperature_nominal_value=1  temperature_nominal_unit=K  x_backlash_specify=off  x_backlash_priority=None  x_backlash=0 mm  x_backlash_nominal_specify=off  x_backlash_nominal_value=1  x_backlash_nominal_unit=mm  f_hardstop_specify=off  f_hardstop_priority=None  f_hardstop=0 N  f_hardstop_nominal_specify=off  f_hardstop_nominal_value=1  f_hardstop_nominal_unit=N  v_backlash_specify=off  v_backlash_priority=None  v_backlash=0 m/s  v_backlash_nominal_specify=off  v_backlash_nominal_value=1  v_backlash_nominal_unit=m/s
  Inertia Kv : fl_lib/Mechanical/Rotational Elements/Inertia  inertia=1 kg*m^2  num_ports=foundation.enum.numPorts2.two  w_specify=off  w_priority=High  w=0 rad/s  w_nominal_specify=off  w_nominal_value=1  w_nominal_unit=rad/s  t_specify=off  t_priority=None  t=0 N*m  t_nominal_specify=off  t_nominal_value=1  t_nominal_unit=N*m
      settings: InternalSimscapePortConfiguration="{\"Bottom\":[],\"Left\":[{\"id\":\"I\",\"label\":\"\",\"type\":\"foundation.mechanical.rotational.rotational\"}],\"Right\":[{\"id\":\"J\",\"label\":\"\",\"type\":\"foundation.mechanical.rotational.rotational\"}],\"Top\":[]}"
  B : PMIOPort  Side=Right
  F : PMIOPort  Port=2  Side=Right
  connections:
  F/RConn1 -- Gear Kv/RConn1
  B/RConn1 -- Inertia Kv/LConn1
  Inertia Kv/RConn1 -- Gear Kv/LConn1

== system sm_wheel_loader_lib/CVT Power Split Hydromechanical/Gears HS In ==
  Gear 1_2 : sdl_lib/Gears/Simple Gear  ratio=HMPST.GearTrain.Gear2.TeethNum/HMPST.GearTrain.Gear1.TeethNum  rotation_direction=3-2*(2)  friction_model=sdl.enum.gear_efficiencies_load.constant  T_noload=0.1 N*m  T_nom=5 N*m  efficiency_nom=0.8  efficiency=0.995  temperature_TLU=[ 280 300 320 ] K  load_TLU=[ 1 5 10 ] N*m  efficiency_TLU=[ 0.95 0.9 0.85 ]  efficiency_TLU2=[ 0.85 0.8 0.75; 0.95 0.9 0.85; 0.85 0.8 0.7 ]  w_thr=0.01 rad/s  pwr_thr=0.001 W  enable_backlash=false  hardstop_model=simscape.enum.hardstop.smooth  backlash_distance=1e-3 mm  r_base=0.1 m  transition=1e-4 mm  backlash_stiffness=1e6 N/m  backlash_damping=1e3 N*s/m  coeff_rest=0.7  v_tol=0.001 m/s  f_tol=0 N  mu_visc=[ 0 0] N*m/(rad/s)  thermal_mass=50 J/K  temperature_specify=off  temperature_priority=High  temperature=300 K  temperature_nominal_specify=off  temperature_nominal_value=1  temperature_nominal_unit=K  x_backlash_specify=off  x_backlash_priority=None  x_backlash=0 mm  x_backlash_nominal_specify=off  x_backlash_nominal_value=1  x_backlash_nominal_unit=mm  f_hardstop_specify=off  f_hardstop_priority=None  f_hardstop=0 N  f_hardstop_nominal_specify=off  f_hardstop_nominal_value=1  f_hardstop_nominal_unit=N  v_backlash_specify=off  v_backlash_priority=None  v_backlash=0 m/s  v_backlash_nominal_specify=off  v_backlash_nominal_value=1  v_backlash_nominal_unit=m/s
  Gear 2_3 : sdl_lib/Gears/Simple Gear  ratio=HMPST.GearTrain.Gear3.TeethNum/HMPST.GearTrain.Gear2.TeethNum  rotation_direction=3-2*(2)  friction_model=sdl.enum.gear_efficiencies_load.constant  T_noload=0.1 N*m  T_nom=5 N*m  efficiency_nom=0.8  efficiency=0.995  temperature_TLU=[ 280 300 320 ] K  load_TLU=[ 1 5 10 ] N*m  efficiency_TLU=[ 0.95 0.9 0.85 ]  efficiency_TLU2=[ 0.85 0.8 0.75; 0.95 0.9 0.85; 0.85 0.8 0.7 ]  w_thr=0.01 rad/s  pwr_thr=0.001 W  enable_backlash=false  hardstop_model=simscape.enum.hardstop.smooth  backlash_distance=1e-3 mm  r_base=0.1 m  transition=1e-4 mm  backlash_stiffness=1e6 N/m  backlash_damping=1e3 N*s/m  coeff_rest=0.7  v_tol=0.001 m/s  f_tol=0 N  mu_visc=[0 0] N*m/(rad/s)  thermal_mass=50 J/K  temperature_specify=off  temperature_priority=High  temperature=300 K  temperature_nominal_specify=off  temperature_nominal_value=1  temperature_nominal_unit=K  x_backlash_specify=off  x_backlash_priority=None  x_backlash=0 mm  x_backlash_nominal_specify=off  x_backlash_nominal_value=1  x_backlash_nominal_unit=mm  f_hardstop_specify=off  f_hardstop_priority=None  f_hardstop=0 N  f_hardstop_nominal_specify=off  f_hardstop_nominal_value=1  f_hardstop_nominal_unit=N  v_backlash_specify=off  v_backlash_priority=None  v_backlash=0 m/s  v_backlash_nominal_specify=off  v_backlash_nominal_value=1  v_backlash_nominal_unit=m/s
  "    E" : PMIOPort  Side=Left
  E : PMIOPort  Port=2  Side=Right
  "    I" : PMIOPort  Port=3  Side=Left
  I : PMIOPort  Port=4  Side=Right
  "    H" : PMIOPort  Port=5  Side=Left
  H : PMIOPort  Port=6  Side=Right
  connections:
  Gear 2_3/RConn1 -- H/RConn1 -- "    H"/RConn1
  Gear 1_2/LConn1 -- E/RConn1 -- "    E"/RConn1
  "    I"/RConn1 -- I/RConn1 -- Gear 2_3/LConn1 -- Gear 1_2/RConn1

== system sm_wheel_loader_lib/CVT Power Split Hydromechanical/Gears HS Out ==
  Gear 4_5 : sdl_lib/Gears/Simple Gear  ratio=HMPST.GearTrain.Gear5.TeethNum/HMPST.GearTrain.Gear4.TeethNum  rotation_direction=3-2*(2)  friction_model=sdl.enum.gear_efficiencies_load.constant  T_noload=0.1 N*m  T_nom=5 N*m  efficiency_nom=0.8  efficiency=0.995  temperature_TLU=[ 280 300 320 ] K  load_TLU=[ 1 5 10 ] N*m  efficiency_TLU=[ 0.95 0.9 0.85 ]  efficiency_TLU2=[ 0.85 0.8 0.75; 0.95 0.9 0.85; 0.85 0.8 0.7 ]  w_thr=0.01 rad/s  pwr_thr=0.001 W  enable_backlash=false  hardstop_model=simscape.enum.hardstop.smooth  backlash_distance=1e-3 mm  r_base=0.1 m  transition=1e-4 mm  backlash_stiffness=1e6 N/m  backlash_damping=1e3 N*s/m  coeff_rest=0.7  v_tol=0.001 m/s  f_tol=0 N  mu_visc=[0 0] N*m/(rad/s)  thermal_mass=50 J/K  temperature_specify=off  temperature_priority=High  temperature=300 K  temperature_nominal_specify=off  temperature_nominal_value=1  temperature_nominal_unit=K  x_backlash_specify=off  x_backlash_priority=None  x_backlash=0 mm  x_backlash_nominal_specify=off  x_backlash_nominal_value=1  x_backlash_nominal_unit=mm  f_hardstop_specify=off  f_hardstop_priority=None  f_hardstop=0 N  f_hardstop_nominal_specify=off  f_hardstop_nominal_value=1  f_hardstop_nominal_unit=N  v_backlash_specify=off  v_backlash_priority=None  v_backlash=0 m/s  v_backlash_nominal_specify=off  v_backlash_nominal_value=1  v_backlash_nominal_unit=m/s
  "    F" : PMIOPort  Side=Left
  F : PMIOPort  Port=2  Side=Right
  "    B" : PMIOPort  Port=3  Side=Left
  B : PMIOPort  Port=4  Side=Right
  connections:
  Gear 4_5/RConn1 -- F/RConn1 -- "    F"/RConn1
  Gear 4_5/LConn1 -- B/RConn1 -- "    B"/RConn1
